simulink model "lab6_task4_model3"  (R2024b)
settings: Solver=ode45  StartTime=0.0  StopTime=10.0  MaxStep=0.01  RelTol=1e-3
settings Model: Creator=Beanie  LastModifiedBy=Beanie

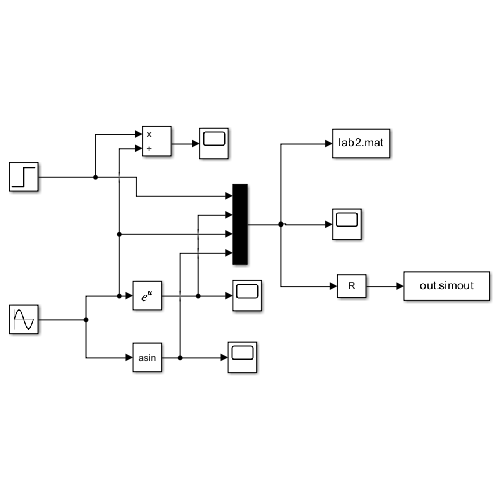
[thumbnail: Simulink's stored preview of the top-level diagram]
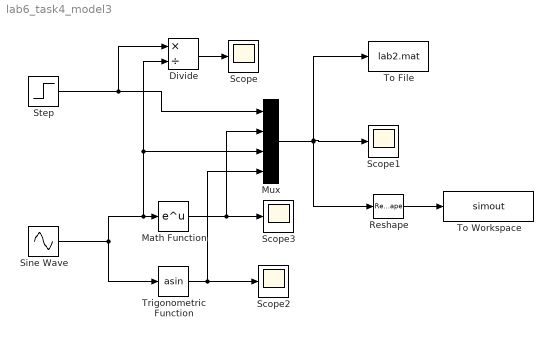
== system lab6_task4_model3 ==
  Divide : Product  Inputs=*/
  Math Function : Math
  Mux : Mux
  Reshape : Reshape  OutputDimensionality=Customize  OutputDimensions=[2 2]
  Scope{,1..3} (4 alike) : Scope
  Sine Wave : Sin  Frequency=2*pi  SampleTime=0
  Step : Step  SampleTime=0
  To File : ToFile  Filename=lab2.mat  SaveFormat=Timeseries
  To Workspace : ToWorkspace  VariableName=simout  SaveFormat=Structure With Time  SampleTime=-1
  Trigonometric Function : Trigonometry  Operator=asin
  wires:
  Step/1 -> Divide/1, Mux/1
  Sine Wave/1 -> Trigonometric Function/1, Mux/3, Divide/2, Math Function/1
  Math Function/1 -> Scope3/1, Mux/2
  Trigonometric Function/1 -> Scope2/1, Mux/4
  Mux/1 -> Reshape/1, Scope1/1, To File/1
  Reshape/1 -> To Workspace/1
  Divide/1 -> Scope/1
